simulink model "Absolute_or_Relative_damping"  (R2025a)
settings: Solver=VariableStepAuto  StartTime=0.0  StopTime=tf  RelTol=1e-3
values from neighbouring files (symbols this model uses):
  dampCase = 2    [init.m]    (also in visu_m.m = evalin('base','dampCase'))
  gamma = k2 / k1    (= 10)    [init.m]    (also in visu_m.m = evalin('base','gamma'))
  K = 1    [init.m]    (also in visu_m.m = evalin('base','K'))
  L = D_mat-W_mat    [init.m]
  x_0 = [x1_0; v1_0;      x2_0; v2_0;      x3_0; v3_0;      x4_0; v4_0;      x5_0; v5_0]    [init.m]
settings Model: Creator=Lenovo  LastModifiedBy=Lenovo
settings DataIOCC: ReturnWorkspaceOutputs=off

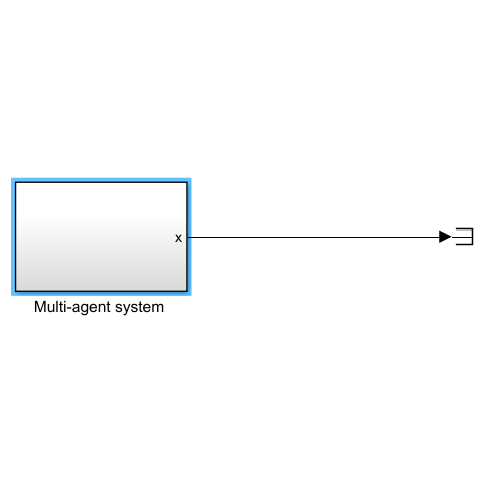
[thumbnail: Simulink's stored preview of the top-level diagram]
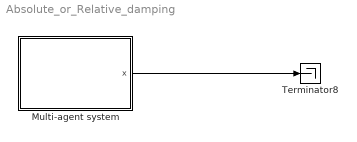
== system Absolute_or_Relative_damping ==
  "Multi-agent system " : Subsystem
  Terminator8 : Terminator
  wires:
  "Multi-agent system "/1(x) -> Terminator8/1

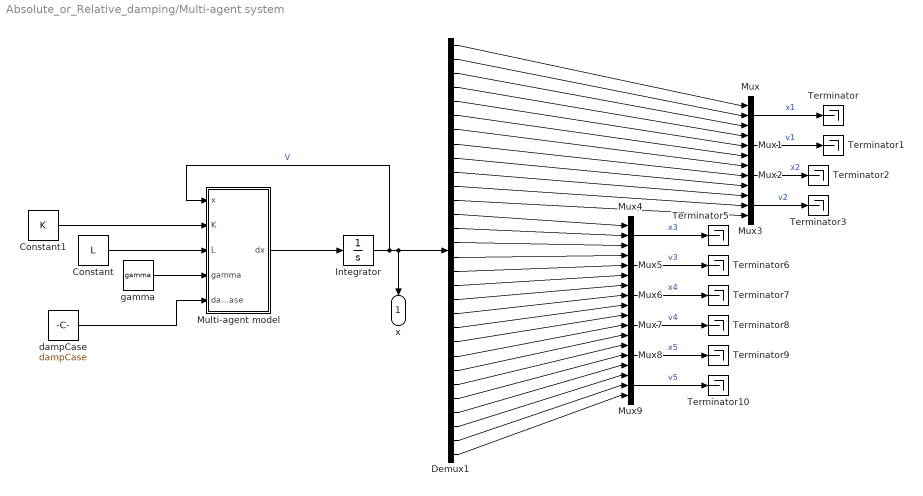
== system Absolute_or_Relative_damping/Multi-agent system  ==
  Constant : Constant  Value=L  OutDataTypeStr=double
  Constant1 : Constant  Value=K
  Demux1 : Demux  Outputs=30
  Integrator : Integrator  InitialCondition=x_0
  Multi-agent model : MATLAB Function  TreatAsAtomicUnit=on
  Mux{,1..9} (10 alike) : Mux  Inputs=3
  Terminator{,1..3,5..10} (10 alike) : Terminator
  dampCase : Constant  Value=dampCase  OutDataTypeStr=double
  gamma : Constant  Value=gamma  OutDataTypeStr=double
  x : Outport  VectorParamsAs1DForOutWhenUnconnected=off
  wires:
  Multi-agent model/1(dx) -> Integrator/1
  Integrator/1 -> x/1, Demux1/1, Multi-agent model/1(x)  "V"
  Constant1/1 -> Multi-agent model/2(K)
  Mux/1 -> Terminator/1  "x1"
  Mux1/1 -> Terminator1/1  "v1"
  Demux1/1 -> Mux/1
  Demux1/2 -> Mux/2
  Demux1/3 -> Mux/3
  Demux1/4 -> Mux1/1
  Demux1/5 -> Mux1/2
  Demux1/6 -> Mux1/3
  Mux2/1 -> Terminator2/1  "x2"
  Demux1/7 -> Mux2/1
  Demux1/8 -> Mux2/2
  Demux1/9 -> Mux2/3
  Mux3/1 -> Terminator3/1  "v2"
  Demux1/10 -> Mux3/1
  Demux1/11 -> Mux3/2
  Demux1/12 -> Mux3/3
  Demux1/13 -> Mux4/1
  Demux1/14 -> Mux4/2
  Demux1/15 -> Mux4/3
  Demux1/16 -> Mux5/1
  Demux1/17 -> Mux5/2
  Demux1/18 -> Mux5/3
  Demux1/19 -> Mux6/1
  Demux1/20 -> Mux6/2
  Demux1/21 -> Mux6/3
  Demux1/22 -> Mux7/1
  Demux1/23 -> Mux7/2
  Demux1/24 -> Mux7/3
  Demux1/25 -> Mux8/1
  Demux1/26 -> Mux8/2
  Demux1/27 -> Mux8/3
  Demux1/28 -> Mux9/1
  Demux1/29 -> Mux9/2
  Demux1/30 -> Mux9/3
  Mux4/1 -> Terminator5/1  "x3"
  Mux5/1 -> Terminator6/1  "v3"
  Mux6/1 -> Terminator7/1  "x4"
  Mux7/1 -> Terminator8/1  "v4"
  Mux8/1 -> Terminator9/1  "x5"
  Mux9/1 -> Terminator10/1  "v5"
  Constant/1 -> Multi-agent model/3(L)
  gamma/1 -> Multi-agent model/4(gamma)
  dampCase/1 -> Multi-agent model/5(dampCase)

== matlab function Absolute_or_Relative_damping/Multi-agent system /Multi-agent model ==
  data: x input; K input; dx output; L input; gamma input; dampCase input
function dx = fcn(x,K,L,gamma,dampCase)

dx = zeros(30,1);

x1 = x(1:3);    v1 = x(4:6);
x2 = x(7:9);    v2 = x(10:12);
x3 = x(13:15);  v3 = x(16:18);
x4 = x(19:21);  v4 = x(22:24);
x5 = x(25:27);  v5 = x(28:30);

X = [x1,x2,x3,x4,x5];
V = [v1,v2,v3,v4,v5];  

Lt = L.';  

posTerm = -K * (X * Lt);     % 3x5


if dampCase == 2
    dampTerm = -gamma * K * (V * Lt);  % 3x5
else
    dampTerm = -gamma * K * V;         % 3x5
end

Vdot = posTerm + dampTerm;             % 3x5

dx(1:3)   = v1;   dx(4:6)   = Vdot(:,1);
dx(7:9)   = v2;   dx(10:12) = Vdot(:,2);
dx(13:15) = v3;   dx(16:18) = Vdot(:,3);
dx(19:21) = v4;   dx(22:24) = Vdot(:,4);
dx(25:27) = v5;   dx(28:30) = Vdot(:,5);

end
